simulink model "RobotDynamicsControl"  (R2026a)
settings: Solver=ode15s  MaxStep=0.6
undefined symbols (not defined in the file or in its folder): scenario, setdiff
libraries: robotcorelib x2, robotmaniplib x2
settings Model: Creator=smaddina  LastModifiedBy=smaddina

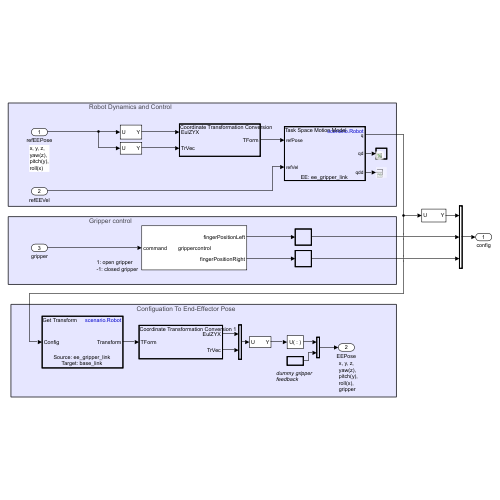
[thumbnail: Simulink's stored preview of the top-level diagram]
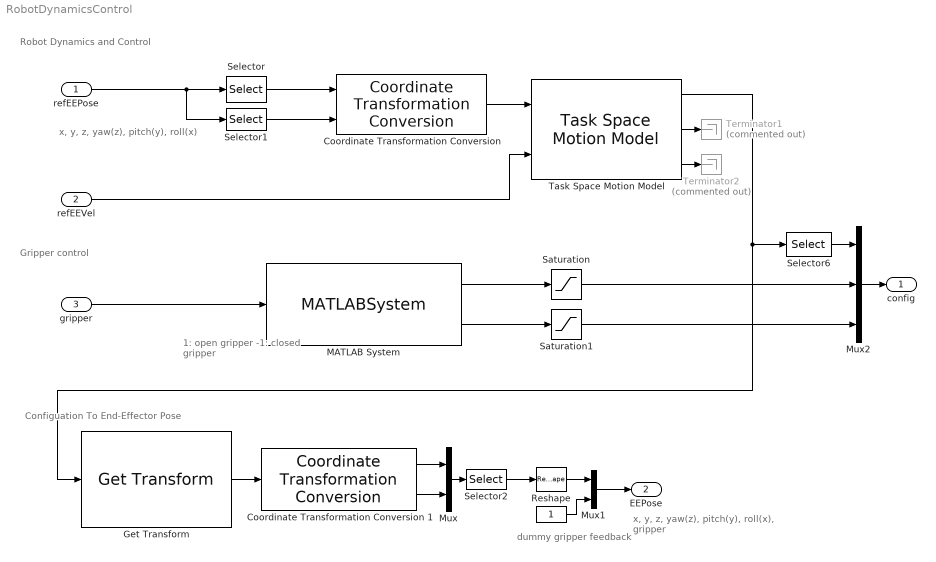
== system RobotDynamicsControl ==
  note: Gripper control
  note: dummy gripper
      | feedback
  note: x, y, z,
      | yaw(z),
      | pitch(y),
      | roll(x)
  note: x, y, z,
      | yaw(z),
      | pitch(y),
      | roll(x),
      | gripper
  note: Configuation To End-Effector Pose
  note: Robot Dynamics and Control
  note: 1: open gripper
      | -1: closed gripper
  refEEPose : Inport  PortDimensions=scenario.NumStates-1  SampleTime=scenario.Ts
  refEEVel : Inport  Port=2  PortDimensions=scenario.NumStates-1
  gripper : Inport  Port=3  PortDimensions=1
  " " : Constant
  Coordinate Transformation Conversion : robotcorelib/Coordinate Transformation Conversion  InputRepresentation=Euler Angles  InputEulerSequence=ZYX  ShowTrVecInputPort=on  OutputRepresentation=Homogeneous Transformation  OutputEulerSequence=ZYX  ShowTrVecOutputPort=on  SimulateUsing=Interpreted execution
  Coordinate Transformation Conversion 1 : robotcorelib/Coordinate Transformation Conversion  InputRepresentation=Homogeneous Transformation  InputEulerSequence=ZYX  ShowTrVecInputPort=on  OutputRepresentation=Euler Angles  OutputEulerSequence=ZYX  ShowTrVecOutputPort=on  SimulateUsing=Interpreted execution
  "Get Transform " : robotmaniplib/Get Transform  RigidBodyTree=scenario.Robot  SourceBody=ee_gripper_link  TargetBody=base_link  SimulateUsing=Interpreted execution
  MATLAB System : MATLABSystem  System=grippercontrol  FingerPositionMin=scenario.FingerPositionMin  FingerPositionMax=scenario.FingerPositionMax  Clearance=0.001  StiffnessKp=1000  DampingKd=200  EffortLimit=60  SimFrequency=500  ControlFrequency=5  SimulateUsing=Code generation
      mask Type: grippercontrol
  Mux : Mux  Inputs=2
  Mux1 : Mux  Inputs=2
  Mux2 : Mux  Inputs=3
  Reshape : Reshape
  Saturation : Saturate  UpperLimit=inf  LowerLimit=max(scenario.FingerClose, scenario.FingerPositionMin)
  Saturation1 : Saturate  UpperLimit=inf  LowerLimit=max(scenario.FingerClose, scenario.FingerPositionMin)
  Selector : Selector  InputPortWidth=scenario.NumStates-1  IndexOptions=Index vector (dialog)  Indices=[4,5,6]  OutputSizes=1
  Selector1 : Selector  InputPortWidth=scenario.NumStates-1  IndexOptions=Index vector (dialog)  Indices=[1,2,3]  OutputSizes=1
  Selector2 : Selector  InputPortWidth=6  IndexOptions=Index vector (dialog)  Indices=[4,5,6,1,2,3]  OutputSizes=1
  Selector6 : Selector  InputPortWidth=scenario.NumConfig  IndexOptions=Index vector (dialog)  Indices=setdiff(1:scenario.NumConfig, scenario.FingerLinkIds)  OutputSizes=1
  "Task Space Motion Model " : robotmaniplib/Task Space Motion Model  RigidBodyTree=scenario.Robot  EndEffector=ee_gripper_link  ProportionalGain=500*eye(6)*2  DerivativeGain=100*eye(6)*2  JointDamping=1  ShowExternalForcePort=off  InitConfig=scenario.RobotInitConfig  InitJointVel=zeros(1, scenario.NumConfig)  SimulateUsing=Interpreted execution
  Terminator1 : Terminator  Commented=on
  Terminator2 : Terminator  Commented=on
  config : Outport
  EEPose : Outport  Port=2
  wires:
  Selector/1 -> Coordinate Transformation Conversion/1
  Selector1/1 -> Coordinate Transformation Conversion/2
  refEEVel/1 -> "Task Space Motion Model "/2
  "Task Space Motion Model "/2 -> Terminator1/1
  "Task Space Motion Model "/3 -> Terminator2/1
  Coordinate Transformation Conversion/1 -> "Task Space Motion Model "/1
  "Task Space Motion Model "/1 -> Selector6/1, "Get Transform "/1
  "Get Transform "/1 -> Coordinate Transformation Conversion 1/1
  Coordinate Transformation Conversion 1/1 -> Mux/1
  Coordinate Transformation Conversion 1/2 -> Mux/2
  Mux/1 -> Selector2/1
  Selector2/1 -> Reshape/1
  Mux2/1 -> config/1
  Selector6/1 -> Mux2/1
  Reshape/1 -> Mux1/1
  " "/1 -> Mux1/2
  Mux1/1 -> EEPose/1
  refEEPose/1 -> Selector1/1, Selector/1
  MATLAB System/1 -> Saturation/1
  MATLAB System/2 -> Saturation1/1
  gripper/1 -> MATLAB System/1
  Saturation/1 -> Mux2/2
  Saturation1/1 -> Mux2/3
